simulink subsystem "Intake_Controls_sub"  (R2023b)
settings: Solver=VariableStepAuto  StartTime=0.0  StopTime=10.0  RelTol=1e-3
undefined symbols (not defined in the file): Rebuilt_Intake_Cycle_Angle_In, Rebuilt_Intake_Cycle_Angle_Out, Rebuilt_Intake_Des_Angle_In, Rebuilt_Intake_Des_Angle_Out, Rebuilt_Intake_Meas_In_Disable, Rebuilt_Intake_Meas_Out_Disable, Rebuilt_Roller_Desired_Speed, Rebuilt_Roller_Error_Integral_Enable, Rebuilt_Roller_Intake_In_Delay, t_sample
libraries: simulink x9, Controls_Components_lib x3
settings Model: Creator=ander  LastModifiedBy=ander

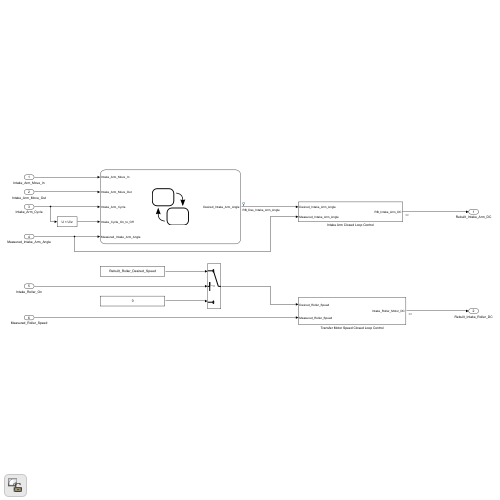
[thumbnail: Simulink's stored preview of the top-level diagram]
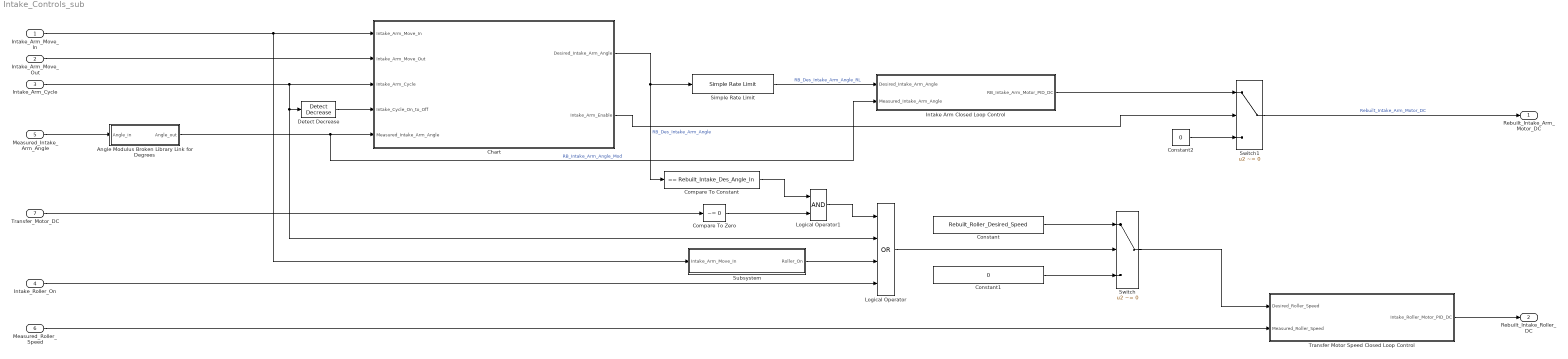
== system Intake_Controls_sub ==
  Intake_Arm_Move_In : Inport
  Intake_Arm_Move_Out : Inport  Port=2
  Intake_Arm_Cycle : Inport  Port=3
  Intake_Roller_On : Inport  Port=4
  Measured_Intake_Arm_Angle : Inport  Port=5
  Measured_Roller_Speed : Inport  Port=6
  Transfer_Motor_DC : Inport  Port=7
  Angle Modulus Broken Library Link for Degrees : Subsystem
  Chart : Stateflow chart  TreatAsAtomicUnit=on
  Compare To Constant : simulink/Logic and Bit Operations/Compare To Constant  relop===  const=Rebuilt_Intake_Des_Angle_In  OutDataTypeStr=boolean
  Compare To Zero : simulink/Logic and Bit Operations/Compare To Zero  relop=~=  OutDataTypeStr=boolean
  Constant : Constant  Value=Rebuilt_Roller_Desired_Speed
  Constant1 : Constant  Value=0
  Constant2 : Constant  Value=0
  Detect Decrease : simulink/Logic and Bit Operations/Detect Decrease  vinit=0.0  OutDataTypeStr=boolean
  Intake Arm Closed Loop Control : Subsystem
  Logical Operator : Logic  Operator=OR  Inputs=4  AllPortsSameDT=off  OutDataTypeStr=boolean
  Logical Operator1 : Logic  AllPortsSameDT=off  OutDataTypeStr=boolean
  Simple Rate Limit : Controls_Components_lib/Simple Rate Limit  Rate_Limit_Inc=Rebuilt_Intake_RL_Inc  Rate_Limit_Dec=Rebuilt_Intake_RL_Dec
  Subsystem : Subsystem
  Switch : Switch  Criteria=u2 ~= 0  SaturateOnIntegerOverflow=off  InputSameDT=off
  Switch1 : Switch  Criteria=u2 ~= 0  SaturateOnIntegerOverflow=off  InputSameDT=off
  Transfer Motor Speed Closed Loop Control : Subsystem
  Rebuilt_Intake_Arm_Motor_DC : Outport
  Rebuilt_Intake_Roller_DC : Outport  Port=2
  wires:
  Intake_Arm_Move_Out/1 -> Chart/2(Intake_Arm_Move_Out)
  Intake_Arm_Move_In/1 -> Subsystem/1(Intake_Arm_Move_In), Chart/1(Intake_Arm_Move_In)
  Intake_Arm_Cycle/1 -> Chart/3(Intake_Arm_Cycle), Detect Decrease/1, Logical Operator/2
  Measured_Intake_Arm_Angle/1 -> Angle Modulus Broken Library Link for Degrees/1(Angle_in)
  Detect Decrease/1 -> Chart/4(Intake_Cycle_On_to_Off)
  Chart/1(Desired_Intake_Arm_Angle) -> Simple Rate Limit/1, Compare To Constant/1  "RB_Des_Intake_Arm_Angle"
  Transfer Motor Speed Closed Loop Control/1(Intake_Roller_Motor_PID_DC) -> Rebuilt_Intake_Roller_DC/1
  Measured_Roller_Speed/1 -> Transfer Motor Speed Closed Loop Control/2(Measured_Roller_Speed)
  Switch/1 -> Transfer Motor Speed Closed Loop Control/1(Desired_Roller_Speed)
  Constant/1 -> Switch/1
  Constant1/1 -> Switch/3
  Simple Rate Limit/1 -> Intake Arm Closed Loop Control/1(Desired_Intake_Arm_Angle)  "RB_Des_Intake_Arm_Angle_RL"
  Angle Modulus Broken Library Link for Degrees/1(Angle_out) -> Chart/5(Measured_Intake_Arm_Angle), Intake Arm Closed Loop Control/2(Measured_Intake_Arm_Angle)  "RB_Intake_Arm_Angle_Mod"
  Intake_Roller_On/1 -> Logical Operator/4
  Logical Operator/1 -> Switch/2
  Subsystem/1(Roller_On) -> Logical Operator/3
  Transfer_Motor_DC/1 -> Compare To Zero/1
  Logical Operator1/1 -> Logical Operator/1
  Compare To Zero/1 -> Logical Operator1/2
  Compare To Constant/1 -> Logical Operator1/1
  Chart/2(Intake_Arm_Enable) -> Switch1/2
  Intake Arm Closed Loop Control/1(RB_Intake_Arm_Motor_PID_DC) -> Switch1/1
  Constant2/1 -> Switch1/3
  Switch1/1 -> Rebuilt_Intake_Arm_Motor_DC/1  "Rebuilt_Intake_Arm_Motor_DC"

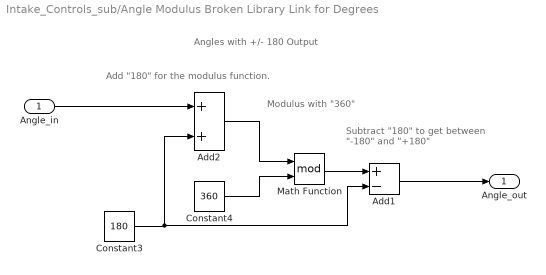
== system Intake_Controls_sub/Angle Modulus Broken Library Link for Degrees ==
  note: Add "180" for the modulus function.
  note: Modulus with "360"
  note: Subtract "180" to get
      | between "-180" and "+180"
  note: Angles with +/- 180 Output
  Angle_in : Inport
  Add1 : Sum  Inputs=+-
  Add2 : Sum
  Constant3 : Constant  Value=180
  Constant4 : Constant  Value=360
  Math Function : Math  Operator=mod
  Angle_out : Outport
  wires:
  Angle_in/1 -> Add2/1
  Constant3/1 -> Add1/2, Add2/2
  Add2/1 -> Math Function/1
  Constant4/1 -> Math Function/2
  Math Function/1 -> Add1/1
  Add1/1 -> Angle_out/1

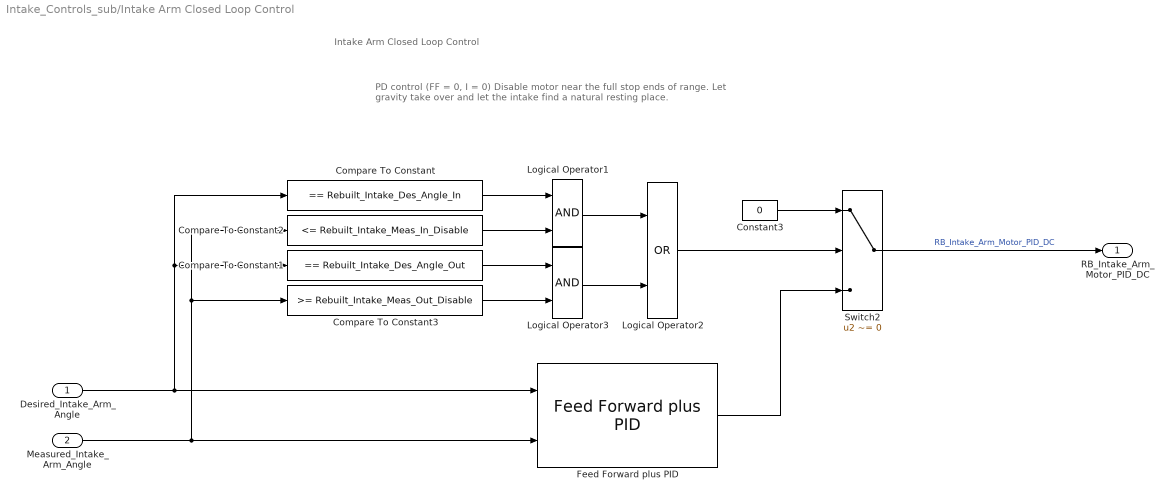
== system Intake_Controls_sub/Intake Arm Closed Loop Control ==
  note: Intake Arm Closed Loop Control
  note: PD control (FF = 0, I = 0)
      | Disable motor near the full stop ends of range.
      | Let gravity take over and let the intake find a natural resting place.
  Desired_Intake_Arm_Angle : Inport
  Measured_Intake_Arm_Angle : Inport  Port=2
  Compare To Constant : simulink/Logic and Bit Operations/Compare To Constant  relop===  const=Rebuilt_Intake_Des_Angle_In  OutDataTypeStr=boolean
  Compare To Constant1 : simulink/Logic and Bit Operations/Compare To Constant  relop===  const=Rebuilt_Intake_Des_Angle_Out  OutDataTypeStr=boolean
  Compare To Constant2 : simulink/Logic and Bit Operations/Compare To Constant  relop=<=  const=Rebuilt_Intake_Meas_In_Disable  OutDataTypeStr=boolean
  Compare To Constant3 : simulink/Logic and Bit Operations/Compare To Constant  relop=>=  const=Rebuilt_Intake_Meas_Out_Disable  OutDataTypeStr=boolean
  Constant3 : Constant  Value=0
  Feed Forward plus PID : Controls_Components_lib/Feed Forward plus PID  Gain_FF=0  Gain_P=Rebuilt_Intake_Arm_Gain_P  Gain_I=0  Gain_D=Rebuilt_Intake_Arm_Gain_D  FilterCoeff_D=0.1  Limit_I_Upper=0.1  Limit_I_Lower=-0.1  Limit_D_Upper=0.1  Limit_D_Lower=-0.1  Limit_T_Upper=1  Limit_T_Lower=-1
  Logical Operator1 : Logic  AllPortsSameDT=off  OutDataTypeStr=boolean
  Logical Operator2 : Logic  Operator=OR  AllPortsSameDT=off  OutDataTypeStr=boolean
  Logical Operator3 : Logic  AllPortsSameDT=off  OutDataTypeStr=boolean
  Switch2 : Switch  Criteria=u2 ~= 0  SaturateOnIntegerOverflow=off  InputSameDT=off
  RB_Intake_Arm_Motor_PID_DC : Outport
  wires:
  Feed Forward plus PID/1 -> Switch2/3
  Constant3/1 -> Switch2/1
  Logical Operator2/1 -> Switch2/2
  Compare To Constant3/1 -> Logical Operator3/2
  Compare To Constant2/1 -> Logical Operator1/2
  Compare To Constant1/1 -> Logical Operator3/1
  Compare To Constant/1 -> Logical Operator1/1
  Logical Operator3/1 -> Logical Operator2/2
  Logical Operator1/1 -> Logical Operator2/1
  Switch2/1 -> RB_Intake_Arm_Motor_PID_DC/1  "RB_Intake_Arm_Motor_PID_DC"
  Measured_Intake_Arm_Angle/1 -> Feed Forward plus PID/2, Compare To Constant3/1, Compare To Constant2/1
  Desired_Intake_Arm_Angle/1 -> Compare To Constant1/1, Compare To Constant/1, Feed Forward plus PID/1

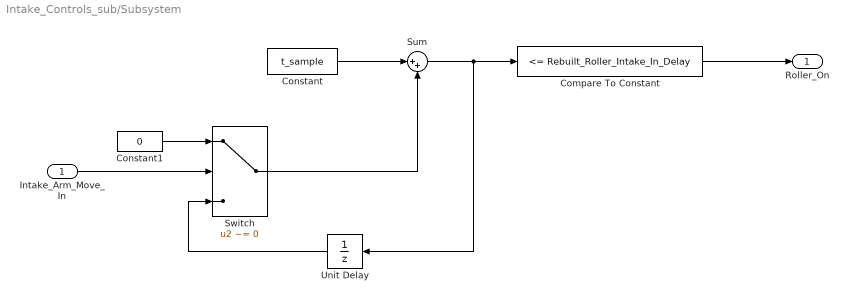
== system Intake_Controls_sub/Subsystem ==
  Intake_Arm_Move_In : Inport
  Compare To Constant : simulink/Logic and Bit Operations/Compare To Constant  relop=<=  const=Rebuilt_Roller_Intake_In_Delay  OutDataTypeStr=boolean
  Constant : Constant  Value=t_sample
  Constant1 : Constant  Value=0
  Sum : Sum  Inputs=|++
  Switch : Switch  Criteria=u2 ~= 0  SaturateOnIntegerOverflow=off  InputSameDT=off
  Unit Delay : UnitDelay  SampleTime=-1  HasFrameUpgradeWarning=on
  Roller_On : Outport
  wires:
  Switch/1 -> Sum/2
  Unit Delay/1 -> Switch/3
  Constant1/1 -> Switch/1
  Intake_Arm_Move_In/1 -> Switch/2
  Compare To Constant/1 -> Roller_On/1
  Sum/1 -> Unit Delay/1, Compare To Constant/1
  Constant/1 -> Sum/1

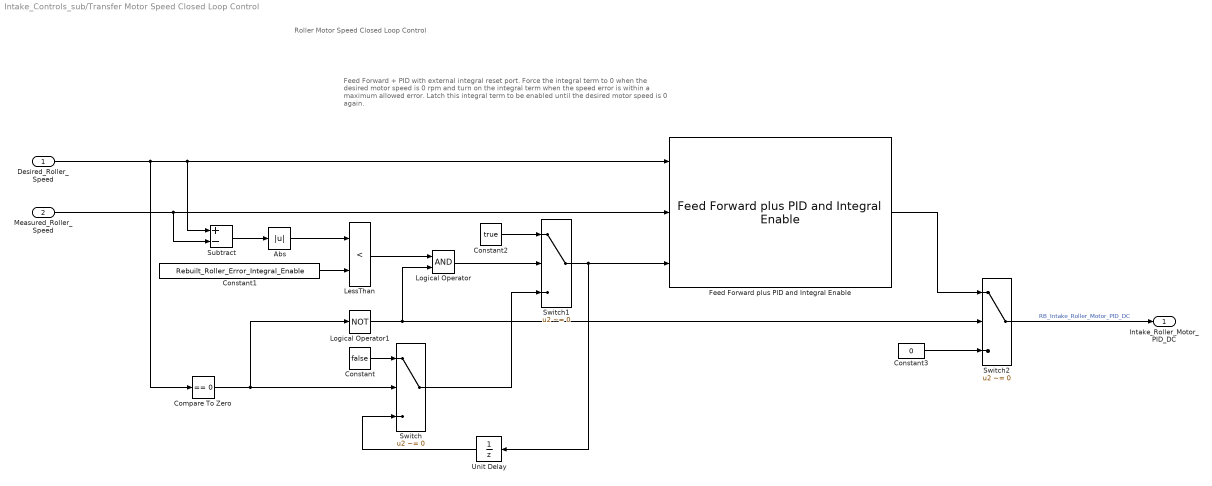
== system Intake_Controls_sub/Transfer Motor Speed Closed Loop Control ==
  note: Roller Motor Speed Closed Loop Control
  note: Feed Forward + PID with external integral reset port.
      |
      | Force the integral term to 0 when the desired motor speed is 0 rpm and turn on the integral term when the speed error is within a maximum allowed error.  Latch this integral term to be enabled until the desired motor speed is 0 again.
  Desired_Roller_Speed : Inport
  Measured_Roller_Speed : Inport  Port=2
  Abs : Abs  SaturateOnIntegerOverflow=off
  Compare To Zero : simulink/Logic and Bit Operations/Compare To Zero  relop===  OutDataTypeStr=boolean
  Constant : Constant  Value=false
  Constant1 : Constant  Value=Rebuilt_Roller_Error_Integral_Enable
  Constant2 : Constant  Value=true
  Constant3 : Constant  Value=0
  Feed Forward plus PID and Integral Enable : Controls_Components_lib/Feed Forward plus PID and Integral Enable  Gain_FF=Rebuilt_Roller_Motor_Gain_FF  Gain_P=Rebuilt_Roller_Motor_Gain_P  Gain_I=Rebuilt_Roller_Motor_Gain_I  Gain_D=0  FilterCoeff_D=0.1  Limit_I_Upper=0.1  Limit_I_Lower=-0.1  Limit_D_Upper=0.1  Limit_D_Lower=-0.1  Limit_T_Upper=1  Limit_T_Lower=-1
  LessThan : RelationalOperator  Operator=<  OutDataTypeStr=boolean  RndMeth=Simplest  InputSameDT=off
  Logical Operator : Logic  AllPortsSameDT=off  OutDataTypeStr=boolean
  Logical Operator1 : Logic  Operator=NOT  AllPortsSameDT=off  OutDataTypeStr=boolean
  Subtract : Sum  Inputs=+-
  Switch : Switch  Criteria=u2 ~= 0  SaturateOnIntegerOverflow=off  InputSameDT=off
  Switch1 : Switch  Criteria=u2 ~= 0  SaturateOnIntegerOverflow=off  InputSameDT=off
  Switch2 : Switch  Criteria=u2 ~= 0  SaturateOnIntegerOverflow=off  InputSameDT=off
  Unit Delay : UnitDelay  SampleTime=-1  HasFrameUpgradeWarning=on
  Intake_Roller_Motor_PID_DC : Outport
  wires:
  Feed Forward plus PID and Integral Enable/1 -> Switch2/1
  Switch2/1 -> Intake_Roller_Motor_PID_DC/1  "RB_Intake_Roller_Motor_PID_DC"
  Constant3/1 -> Switch2/3
  Unit Delay/1 -> Switch/3
  Switch/1 -> Switch1/3
  Switch1/1 -> Feed Forward plus PID and Integral Enable/3, Unit Delay/1
  Constant2/1 -> Switch1/1
  Constant/1 -> Switch/1
  Compare To Zero/1 -> Logical Operator1/1, Switch/2
  Desired_Roller_Speed/1 -> Subtract/1, Feed Forward plus PID and Integral Enable/1, Compare To Zero/1
  Measured_Roller_Speed/1 -> Feed Forward plus PID and Integral Enable/2, Subtract/2
  Abs/1 -> LessThan/1
  Constant1/1 -> LessThan/2
  Subtract/1 -> Abs/1
  LessThan/1 -> Logical Operator/1
  Logical Operator/1 -> Switch1/2
  Logical Operator1/1 -> Switch2/2, Logical Operator/2

== stateflow chart Intake_Controls_sub/Chart ==
  state Wait_for_Button
    entry: Desired_Intake_Arm_Angle = Measured_Intake_Arm_Angle;
    Intake_Arm_Enable = false;
  state Move_Intake_Arm_In
    entry: Desired_Intake_Arm_Angle = Rebuilt_Intake_Des_Angle_In;
    Intake_Arm_Enable = true;
  state Move_Intake_Arm_Out
    entry: Desired_Intake_Arm_Angle = Rebuilt_Intake_Des_Angle_Out;
    Intake_Arm_Enable = true;
  (default) -> Wait_for_Button
  Wait_for_Button -> Move_Intake_Arm_In [order 1] : [Intake_Arm_Move_In || ...
      | Intake_Arm_Cycle]
  Wait_for_Button -> Move_Intake_Arm_Out [order 2] : [Intake_Arm_Move_Out || ...
      | Intake_Arm_Cycle]
  Move_Intake_Arm_In -> Move_Intake_Arm_Out : [Intake_Arm_Move_Out || ...
      | (Intake_Arm_Cycle && ...
      | Measured_Intake_Arm_Angle < ...
      | Rebuilt_Intake_Cycle_Angle_In) || ...
      | Intake_Cycle_On_to_Off]
  Move_Intake_Arm_Out -> Move_Intake_Arm_In : [Intake_Arm_Move_In || ...
      | (Intake_Arm_Cycle && ...
      | Measured_Intake_Arm_Angle > ...
      | Rebuilt_Intake_Cycle_Angle_Out)]
  data: Intake_Arm_Move_In input; Intake_Arm_Move_Out input; Intake_Arm_Cycle input; Intake_Cycle_On_to_Off input; Measured_Intake_Arm_Angle input; Desired_Intake_Arm_Angle output; Rebuilt_Intake_Cycle_Angle_In parameter; Rebuilt_Intake_Des_Angle_Out parameter; Rebuilt_Intake_Des_Angle_In parameter; Rebuilt_Intake_Cycle_Angle_Out parameter; Intake_Arm_Enable output boolean
